simulink library "Steer_Rack_WheelByWire"  (R2025a)
settings: Solver=VariableStepAuto  StartTime=0.0  StopTime=10.0  RelTol=1e-3
undefined symbols (not defined in the file): Steer, Visual, X, Y, Z
libraries: fl_lib x15, sm_lib x11, nesl_utility x10, ee_lib x2, Driver_Systems x1, simulink_extras x1, sdl_lib x1, SteeringWheel x1, Vehicle_Inputs x1
Description:
  | Component of Simscape Vehicle Templates Library
  | 
  | Copyright 2018-2026 The MathWorks, Inc.
settings Model: Creator=smiller  LastModifiedBy=smiller
settings OptimizationCC: ReuseModelBlockBuffer=off
settings ModelReferenceCC: EnableRefExpFcnMdlSchedulingChecks=on
settings RTWCC: GPUComputeCapability=3.5

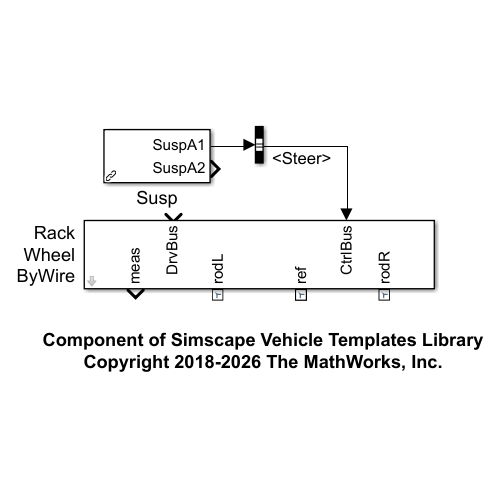
[thumbnail: Simulink's stored preview of the top-level diagram]
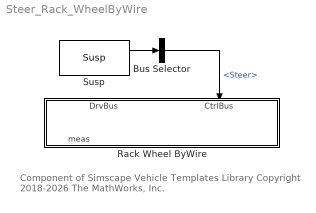
== system Steer_Rack_WheelByWire ==
  note: Component of Simscape Vehicle Templates Library
      | Copyright 2018-2026 The MathWorks, Inc.
  Bus Selector : BusSelector  OutputSignals=Steer
  Rack Wheel ByWire : Subsystem  Tag=PublishSubsystem  VariantControl=Rack  mask(Steer by Wire with Rack Actuation){hp_wheel=Steer.Wheel.sMount.Value, wheel_axis_incl=Steer.Wheel.aAxis.Value, hp_mt_rack=Steer.Rack.sMount.Value, hp_out_rack=Steer.Rack.sOutboard.Value, Wheel=Steer.Wheel, rack_mass=Steer.Rack.m.Value, whl2rack_filter=1/Steer.Rack.fActuatorCutoff.Value, clr_rack=Visual.SteeringRack.clr, opc_rack=Visual.part.opc, radius_rack=Visual.SteeringRack.rad, clr_connhp=Visual.hp.clr, opc_connhp=Visual.hp.opc, size_connhp=Visual.hp.rad, clr_wheel=Visual.SteeringWheel.clr, opc_wheel=Visual.part.opc, DriverHuman=Steer.DriverHuman, Kp_breakpoints=Steer.Control.KpTable.xRack.Value, Kp_values=Steer.Control.KpTable.Kp.Value, Ki=Steer.Control.Ki.Value, Kd=Steer.Control.Kd.Value, tFilt_xRack=1/Steer.Control.fRackxCutoff.Value, tFilt_deriv=1/Steer.Control.fErrDerCutoff.Value, nTrqSteer=Steer.Control.nSteerTrq.Value, vDC=Steer.vMotor.Value, mSteer_trq=Steer.MotorSteer.TorqueSpd.trq.Value, mSteer_spd=Steer.MotorSteer.TorqueSpd.w.Value, mSteer_tc=1/Steer.MotorSteer.fActuatorCutoff.Value, mSteer_J=Steer.MotorSteer.J.Value, mSteer_d=Steer.MotorSteer.D.Value, mRack_trq=Steer.MotorRack.TorqueSpd.trq.Value, mRack_spd=Steer.MotorRack.TorqueSpd.w.Value, mRack_tc=1/Steer.MotorRack.fActuatorCutoff.Value, mRack_J=Steer.MotorRack.J.Value, mRack_d=Steer.MotorRack.D.Value, kRackCompliance=Steer.Rack.kCompliance.Value, DRackCompliance=Steer.Rack.DCompliance.Value, rPinion=Steer.Rack.xPinionRadius.Value, DRack=Steer.Rack.DHousing.Value}
      mask prompts: hp_wheel "HP Wheel [xyz] (m)"; wheel_axis_incl "Wheel Axis Angle (rad)"; hp_mt_rack "HP Rack Mount [xyz] (m)"; hp_out_rack "HP Track Rod Inboard [xyz] (m)"; whl2rack_filter "Rack Motion Filter (sec)"; DriverHuman "Driver Human (structure)"; Kp_breakpoints "Kp Table, Rack position (m)"; Kp_values "Kp Table, Value"; Ki "Ki Controller Gain"; Kd "Kd Controller Gain"; tFilt_xRack "Rack Position Filter (sec)"; tFilt_deriv "Error Derivative Filter (sec)"; nTrqSteer "Gain, Steer Torque"; vDC "DC Voltage (V)"; mSteer_trq "Max Torque (N*m)"; mSteer_spd "Speeds (rpm)"; mSteer_tc "Torque Control Filter (sec)"; mSteer_J "Rotor Inertia (kg*m^2)"; mSteer_d "Rotor Damping (N*m/(m/s))"; mRack_trq "Max Torque (N*m)"; mRack_spd "Speeds (rpm)"; mRack_tc "Torque Control Filter (sec)"; mRack_J "Rotor Inertia (kg*m^2)"; mRack_d "Rotor Damping (N*m/(m/s))"; kRackCompliance "Rack Compliance Stiffness (N/m)"; DRackCompliance "Rack Compliance Damping (N/(m/s))"; rPinion "Pinion Radius (m)"; DRack "Rack Damping (N/(m/s))"
      mask help: Models steer by wire system. Steering wheel angle follows the target angle. Rack position is controlled by a motor The controller also commands a separate motor which applies torque to the steering wheel. This torque provides feedback to the driver concerning the force required to position the rack.
      mask TypeOptions hp_wheel:
      | Ref to Wheel/Transform
      | HP Wheel/TranslationCartesianOffset
      mask TypeOptions hp_mt_rack:
      | Ref to Rack/Transform
      | HP Rack/TranslationCartesianOffset
      mask TypeOptions hp_out_rack: Rack/hp_out
      mask TypeOptions rack_mass: Rack/rack_mass
      mask TypeOptions whl2rack_filter: Physical Signal/InputFilterTimeConstant
      mask TypeOptions clr_rack: Rack/clr_rack
      mask TypeOptions opc_rack: Rack/opc_rack
      mask TypeOptions radius_rack: Rack/radius_rack
      mask TypeOptions clr_connhp:
      | Ref to Rack/Vis
      | Rack
      | Housing/GraphicDiffuseColor
      mask TypeOptions opc_connhp:
      | Ref to Rack/Vis
      | Rack
      | Housing/GraphicOpacity
      mask TypeOptions size_connhp:
      | Ref to Rack/Vis
      | Rack
      | Housing/SphereRadius
      mask TypeOptions clr_wheel: Wheel/clr_wheel
      mask TypeOptions opc_wheel: Wheel/opc_wheel
      mask TypeOptions Kp_breakpoints: Motors/Kp_breakpoints
      mask TypeOptions Kp_values: Motors/Kp_values
      mask TypeOptions Ki: Motors/Ki
      mask TypeOptions Kd: Motors/Kd
      mask TypeOptions tFilt_xRack: Motors/tFilt_xRack
      mask TypeOptions tFilt_deriv: Motors/tFilt_deriv
      mask TypeOptions nTrqSteer: Motors/nTrqSteer
      mask TypeOptions vDC: Motors/vDC
      mask TypeOptions mSteer_trq: Motors/mSteer_trq
      mask TypeOptions mSteer_spd: Motors/mSteer_spd
      mask TypeOptions mSteer_tc: Motors/mSteer_tc
      mask TypeOptions mSteer_J: Motors/mSteer_J
      mask TypeOptions mSteer_d: Motors/mSteer_d
      mask TypeOptions mRack_trq: Motors/mRack_trq
      mask TypeOptions mRack_spd: Motors/mRack_spd
      mask TypeOptions mRack_tc: Motors/mRack_tc
      mask TypeOptions mRack_J: Motors/mRack_J
      mask TypeOptions mRack_d: Motors/mRack_d
      mask TypeOptions kRackCompliance: Motors/kRackCompliance
      mask TypeOptions DRackCompliance: Motors/DRackCompliance
      mask TypeOptions rPinion: Motors/rPinion
      mask TypeOptions DRack: Motors/DRack
      mask DialogControl cont_steer Prompt: Steer
      mask DialogControl grp_strparts Prompt: Parts
      mask DialogControl text_strparts_len Prompt: Length/Radius (m)
      mask DialogControl text_strparts_mass Prompt: Mass (kg)
      mask DialogControl text_strparts_wheel Prompt: Wheel
      mask DialogControl text_strparts_wheel_m Prompt: <CAD file>
      mask DialogControl text_strparts_rack Prompt: Rack
      mask DialogControl text_strparts_rack_len Prompt: <HP Rod Inboard>
      mask DialogControl grp_whl2rack Prompt: Wheel to Rack
      mask DialogControl cont_vis_steer Prompt: Visualization
      mask DialogControl text_steer_vis_clr Prompt: Color [RGB]
      mask DialogControl text_steer_vis_opc Prompt: Opac. (0-1)
      mask DialogControl text_steer_vis_size Prompt: Size (m)
      mask DialogControl text_steer_vis_rack Prompt: Rack
      mask DialogControl text_steer_vis_connhp Prompt: Connections, HP
      mask DialogControl text_steer_vis_wheel Prompt: Wheel
      mask DialogControl text_wheel_size Prompt: <CAD File>
      mask DialogControl cont_driver_human Prompt: Driver Human
      mask DialogControl cont_controller Prompt: Control
      mask DialogControl cont_motor Prompt: Motor
      mask DialogControl grp_steer Prompt: Steer
      mask DialogControl grp_rack Prompt: Rack
      mask DialogControl cont_rack Prompt: Rack
  Susp : Vehicle_Inputs/Control Bus/Susp  SystemSampleTime=-1  VariantActivationTime=update diagram  EmptyChoice=off  PassThrough=off  PassThroughVariantControl=(default)  EmptyChoiceVariantControl=(default)  AllowFlexibleInterface=on  Latency=0  AutoFrameSizeCalculation=off
  wires:
  Bus Selector/1 -> Rack Wheel ByWire/2(CtrlBus)  "<Steer>"
  Susp/1 -> Bus Selector/1

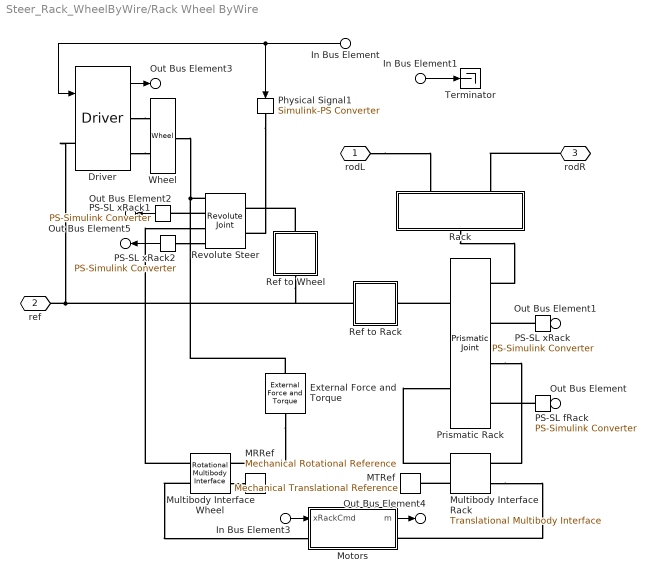
== system Steer_Rack_WheelByWire/Rack Wheel ByWire ==
  In Bus Element1 : Inport  PortName=DrvBus  Element=aSteerWheel
  In Bus Element : Inport  Port=2  PortName=CtrlBus  Element=aSteerWheel
  In Bus Element3 : Inport  Port=2  PortName=CtrlBus  Element=xRack
  Driver : Driver_Systems/Driver  LabelModeActiveChoice=Human  DriverHuman=DriverHuman  VariantLabel=DriverHuman.class.Value
      settings: AttributesFormatString=%<LabelModeActiveChoice>
  External Force and Torque : sm_lib/Forces and Torques/External Force and Torque  EnableForceX=off  EnableForceY=off  EnableForceZ=off  EnableForce=off  ForceResolutionFrame=AttachedFrame  EnableTorqueX=off  EnableTorqueY=off  EnableTorqueZ=on  EnableTorque=off  TorqueResolutionFrame=AttachedFrame
  MRRef : fl_lib/Mechanical/Rotational Elements/Mechanical Rotational Reference
  MTRef : fl_lib/Mechanical/Translational Elements/Mechanical Translational Reference
  Motors : Subsystem  mask{Kp_breakpoints=Kp_breakpoints, Kp_values=Kp_values, Ki=Ki, Kd=Kd, tFilt_deriv=tFilt_deriv, tFilt_xRack=tFilt_xRack, nTrqSteer=nTrqSteer, vDC=vDC, mSteer_trq=mSteer_trq, mSteer_spd=mSteer_spd, mSteer_tc=mSteer_tc, mSteer_J=mSteer_J, mSteer_d=mSteer_d, mRack_trq=mRack_trq, mRack_spd=mRack_spd, mRack_tc=mRack_tc, mRack_J=mRack_J, mRack_d=mRack_d, rPinion=rPinion, kRackCompliance=kRackCompliance, DRackCompliance=DRackCompliance, DRack=DRack}
      mask prompts: Kp_breakpoints "Kp Table, Rack position (m)"; Kp_values "Kp Table, Value"; Ki "Ki Controller Gain"; Kd "Kd Controller Gain"; tFilt_deriv "Filter Constant, Error Derivative"; tFilt_xRack "Filter Constant Rack Position"; nTrqSteer "Gain, Steer Torque"; vDC "DC Voltage (V)"; mSteer_trq "Max Torque (N*m)"; mSteer_spd "Speeds (rpm)"; mSteer_tc "Torque control time constant (sec)"; mSteer_J "Rotor Inertia (kg*m^2)"; mSteer_d "Rotor damping"; mRack_trq "Max Torque (N*m)"; mRack_spd "Speeds (rpm)"; mRack_tc "Torque control time constant (sec)"; mRack_J "Rotor Inertia (kg*m^2)"; mRack_d "Rotor damping"; rPinion "Pinion Radius (m)"; kRackCompliance "Rack Compliance Stiffness (N/m)"; DRackCompliance "Rack Compliance Damping (N/(m/s))"; DRack "Rack Damping (N/(m/s))"
      mask TypeOptions Kp_breakpoints: Control/Kp_breakpoints
      mask TypeOptions Kp_values: Control/Kp_values
      mask TypeOptions Ki: Control/Ki
      mask TypeOptions Kd: Control/Kd
      mask TypeOptions tFilt_deriv: Control/tFilt_deriv
      mask TypeOptions tFilt_xRack: Control/tFilt_xRack
      mask TypeOptions nTrqSteer: Control/nTrqSteer
      mask TypeOptions vDC:
      | DC
      | Voltage
      | Source/v0
      mask TypeOptions mSteer_trq:
      | Motor
      | Steer/T_t
      mask TypeOptions mSteer_spd:
      | Motor
      | Steer/w_t
      mask TypeOptions mSteer_tc:
      | Motor
      | Steer/Tc
      mask TypeOptions mSteer_J:
      | Motor
      | Steer/J
      mask TypeOptions mSteer_d:
      | Motor
      | Steer/lam
      mask TypeOptions mRack_trq:
      | Motor
      | Rack/T_t
      mask TypeOptions mRack_spd:
      | Motor
      | Rack/w_t
      mask TypeOptions mRack_tc:
      | Motor
      | Rack/Tc
      mask TypeOptions mRack_J:
      | Motor
      | Rack/J
      mask TypeOptions mRack_d:
      | Motor
      | Rack/lam
      mask TypeOptions rPinion: Wheel and Axle/R
      mask TypeOptions kRackCompliance:
      | Compliance
      | Spring/spr_rate
      mask TypeOptions DRackCompliance:
      | Compliance
      | Damper/D
      mask TypeOptions DRack: Rack Damper/D
      mask DialogControl tab_control Prompt: Control
      mask DialogControl tab_motor Prompt: Motor
      mask DialogControl grp_steer Prompt: Steer
      mask DialogControl grp_rack Prompt: Rack
      mask DialogControl cont_rack Prompt: Rack
  Multibody Interface Rack : fl_lib/Mechanical/Multibody Interfaces/Translational Multibody Interface
  Multibody Interface Wheel : fl_lib/Mechanical/Multibody Interfaces/Rotational Multibody Interface
  PS-SL fRack : nesl_utility/PS-Simulink Converter  PhysicalDomain=network_engine_domain  SubClassName=ps_output  LeftPortType=input  RightPortType=output  PseudoPeriodic=off  Frequencies=[]  VectorFormat=1-D array  Unit=1  AffineConversion=off
  PS-SL xRack : nesl_utility/PS-Simulink Converter  PhysicalDomain=network_engine_domain  SubClassName=ps_output  LeftPortType=input  RightPortType=output  PseudoPeriodic=off  Frequencies=[]  VectorFormat=1-D array  Unit=1  AffineConversion=off
  PS-SL xRack1 : nesl_utility/PS-Simulink Converter  PhysicalDomain=network_engine_domain  SubClassName=ps_output  LeftPortType=input  RightPortType=output  PseudoPeriodic=off  Frequencies=[]  VectorFormat=1-D array  Unit=rad  AffineConversion=off
  PS-SL xRack2 : nesl_utility/PS-Simulink Converter  PhysicalDomain=network_engine_domain  SubClassName=ps_output  LeftPortType=input  RightPortType=output  PseudoPeriodic=off  Frequencies=[]  VectorFormat=1-D array  Unit=N*m  AffineConversion=off
  Physical Signal1 : nesl_utility/Simulink-PS Converter  PhysicalDomain=network_engine_domain  SubClassName=ps_input  LeftPortType=input  RightPortType=output  PseudoPeriodic=off  Frequencies=[]  NoiseDistribution=none  NoiseParameters=[]  Unit=rad  AffineConversion=off  FilteringAndDerivatives=filter  SimscapeFilterOrder=2  InputFilterTimeConstant=whl2rack_filter  UdotUserProvided=0
      settings: AttributesFormatString=|
      | Filter Time Constant
      | %<InputFilterTimeConstant> sec
  Prismatic Rack : sm_lib/Joints/Prismatic Joint  JointMode=Normal  CompositeWrenchDir=FollowerOnBase  CompositeWrenchFrame=BaseFrame  SenseConstraintForce=off  SenseConstraintTorque=off  SenseTotalForce=off  SenseTotalTorque=off  PositionTargetSpecify=on  PositionTargetPriority=Low  PositionTargetValue=0  PositionTargetValueUnits=m  VelocityTargetSpecify=off  VelocityTargetPriority=High  VelocityTargetValue=0  VelocityTargetValueUnits=m/s  EquilibriumPosition=0  EquilibriumPositionUnits=m  SpringStiffness=0  SpringStiffnessUnits=N/m  DampingCoefficient=1e2*0  DampingCoefficientUnits=N/(m/s)  LowerLimitSpecify=off  LowerLimitBound=-1  LowerLimitBoundUnits=m  LowerLimitStiffness=1e6  LowerLimitStiffnessUnits=N/m  LowerLimitDamping=1e3  LowerLimitDampingUnits=N/(m/s)  LowerLimitTransitionRegionWidth=1e-4  LowerLimitTransitionRegionWidthUnits=m  UpperLimitSpecify=off  UpperLimitBound=1  UpperLimitBoundUnits=m  UpperLimitStiffness=1e6  UpperLimitStiffnessUnits=N/m  UpperLimitDamping=1e3  UpperLimitDampingUnits=N/(m/s)  UpperLimitTransitionRegionWidth=1e-4  UpperLimitTransitionRegionWidthUnits=m  TorqueActuationMode=InputTorque  MotionActuationMode=ComputedMotion  SensePosition=on  SenseVelocity=on  SenseAcceleration=off  SenseTorqueForce=on  SenseLowerLimitTorqueForce=off  SenseUpperLimitTorqueForce=off
  Rack : Subsystem  mask{hp_out=hp_out_rack, rack_mass=rack_mass, clr_rack=clr_rack, opc_rack=opc_rack, radius_rack=radius_rack}
      mask prompts: hp_out "HP Track Rod Inboard [xyz] (m)"; rack_mass "Mass (kg)"
      mask init:
      | rack_length = norm(hp_out-hp_out.*[1 -1 1]);
      mask TypeOptions rack_mass: Rack/Mass
      mask TypeOptions clr_rack: Rack/GraphicDiffuseColor
      mask TypeOptions opc_rack: Rack/GraphicOpacity
      mask TypeOptions radius_rack: Rack/CylinderRadius
      mask DialogControl cont_rack Prompt: Rack
      mask DialogControl text_rack_clr Prompt: Color [RGB]
      mask DialogControl text_rack_opc Prompt: Opac. (0-1)
      mask DialogControl text_rack_size Prompt: Size (m)
      mask DialogControl text_rack_rack Prompt: Rack
  Ref to Rack : Subsystem
  Ref to Wheel : Subsystem
  Revolute Steer : sm_lib/Joints/Revolute Joint  JointMode=Normal  CompositeWrenchDir=FollowerOnBase  CompositeWrenchFrame=BaseFrame  SenseConstraintForce=off  SenseConstraintTorque=off  SenseTotalForce=off  SenseTotalTorque=off  PositionTargetSpecify=on  PositionTargetPriority=High  PositionTargetValue=0  PositionTargetValueUnits=deg  VelocityTargetSpecify=off  VelocityTargetPriority=High  VelocityTargetValue=0  VelocityTargetValueUnits=deg/s  EquilibriumPosition=0  EquilibriumPositionUnits=deg  SpringStiffness=0  SpringStiffnessUnits=N*m/deg  DampingCoefficient=0  DampingCoefficientUnits=N*m/(deg/s)  LowerLimitSpecify=off  LowerLimitBound=-90  LowerLimitBoundUnits=deg  LowerLimitStiffness=1e4  LowerLimitStiffnessUnits=N*m/deg  LowerLimitDamping=10  LowerLimitDampingUnits=N*m/(deg/s)  LowerLimitTransitionRegionWidth=0.1  LowerLimitTransitionRegionWidthUnits=deg  UpperLimitSpecify=off  UpperLimitBound=90  UpperLimitBoundUnits=deg  UpperLimitStiffness=1e4  UpperLimitStiffnessUnits=N*m/deg  UpperLimitDamping=10  UpperLimitDampingUnits=N*m/(deg/s)  UpperLimitTransitionRegionWidth=0.1  UpperLimitTransitionRegionWidthUnits=deg  TorqueActuationMode=ComputedTorque  MotionActuationMode=InputMotion  SensePosition=on  SenseVelocity=on  SenseAcceleration=off  SenseTorqueForce=on  SenseLowerLimitTorqueForce=off  SenseUpperLimitTorqueForce=off
  Terminator : Terminator
  Wheel : SteeringWheel/Wheel  LabelModeActiveChoice=Sedan  VariantLabel=Wheel.class.Value
  rodL : PMIOPort  Side=Right
  ref : PMIOPort  Port=2  Side=Right
  rodR : PMIOPort  Port=3  Side=Right
  Out Bus Element : Outport  VectorParamsAs1DForOutWhenUnconnected=off  PortName=meas  Element=FRack
  Out Bus Element1 : Outport  VectorParamsAs1DForOutWhenUnconnected=off  PortName=meas  Element=xRack
  Out Bus Element2 : Outport  VectorParamsAs1DForOutWhenUnconnected=off  PortName=meas  Element=aWheel
  Out Bus Element3 : Outport  VectorParamsAs1DForOutWhenUnconnected=off  PortName=meas  Element=Driver
  Out Bus Element4 : Outport  VectorParamsAs1DForOutWhenUnconnected=off  PortName=meas  Element=Motor
  Out Bus Element5 : Outport  VectorParamsAs1DForOutWhenUnconnected=off  PortName=meas  Element=trqWheel
  wires:
  In Bus Element1/1 -> Terminator/1
  Driver/1 -> Out Bus Element3/1
  PS-SL xRack1/1 -> Out Bus Element2/1
  In Bus Element/1 -> Driver/1, Physical Signal1/1
  PS-SL fRack/1 -> Out Bus Element/1
  PS-SL xRack/1 -> Out Bus Element1/1
  In Bus Element3/1 -> Motors/1(xRackCmd)
  Motors/1(m) -> Out Bus Element4/1
  PS-SL xRack2/1 -> Out Bus Element5/1
  connections:
  Driver/RConn2 -- Wheel/RConn2
  Driver/RConn1 -- Wheel/RConn1
  Multibody Interface Wheel/RConn1 -- Revolute Steer/RConn3
  rodR/RConn1 -- Rack/LConn2
  rodL/RConn1 -- Rack/LConn1
  Prismatic Rack/LConn1 -- Ref to Rack/RConn1
  Ref to Wheel/RConn1 -- Revolute Steer/LConn1
  Wheel/LConn1 -- Revolute Steer/RConn1 -- External Force and Torque/RConn1
  PS-SL xRack/LConn1 -- Prismatic Rack/RConn2
  Rack/RConn1 -- Prismatic Rack/RConn1
  Driver/LConn1 -- ref/RConn1 -- Ref to Rack/LConn1 -- Ref to Wheel/LConn1
  PS-SL fRack/LConn1 -- Prismatic Rack/RConn4
  Multibody Interface Wheel/RConn2 -- Motors/LConn1
  External Force and Torque/LConn1 -- Multibody Interface Wheel/LConn1
  Multibody Interface Wheel/LConn2 -- MRRef/LConn1
  Multibody Interface Rack/RConn2 -- Motors/RConn1
  Prismatic Rack/RConn3 -- Multibody Interface Rack/RConn1
  Multibody Interface Rack/LConn1 -- Prismatic Rack/LConn2
  Multibody Interface Rack/LConn2 -- MTRef/LConn1
  Physical Signal1/RConn1 -- Revolute Steer/LConn2
  Revolute Steer/RConn2 -- PS-SL xRack1/LConn1
  PS-SL xRack2/LConn1 -- Revolute Steer/RConn4

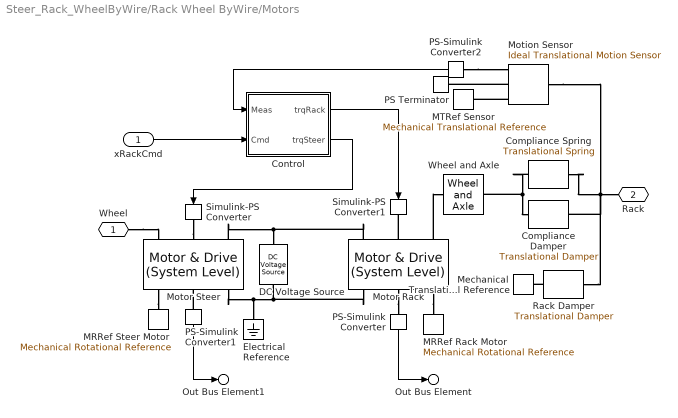
== system Steer_Rack_WheelByWire/Rack Wheel ByWire/Motors ==
  xRackCmd : Inport
  Compliance Damper : fl_lib/Mechanical/Translational Elements/Translational Damper  D=DRackCompliance N*s/m  v_specify=off  v_priority=None  v=0 m/s  v_nominal_specify=off  v_nominal_value=1  v_nominal_unit=m/s  f_specify=off  f_priority=None  f=0 N  f_nominal_specify=off  f_nominal_value=1  f_nominal_unit=N
  Compliance Spring : fl_lib/Mechanical/Translational Elements/Translational Spring  spr_rate=kRackCompliance N/m  v_specify=off  v_priority=None  v=0 m/s  v_nominal_specify=off  v_nominal_value=1  v_nominal_unit=m/s  f_specify=off  f_priority=None  f=0 N  f_nominal_specify=off  f_nominal_value=1  f_nominal_unit=N  x_specify=off  x_priority=High  x=0 m  x_nominal_specify=off  x_nominal_value=1  x_nominal_unit=m
  Control : Subsystem  mask{Kp_breakpoints=Kp_breakpoints, Kp_values=Kp_values, Ki=Ki, Kd=Kd, tFilt_xRack=tFilt_xRack, tFilt_deriv=tFilt_deriv, nTrqSteer=nTrqSteer}
      mask prompts: Kp_breakpoints "Kp Table, Rack position (m)"; Kp_values "Kp Table, Value"; Ki "Ki Controller Gain"; Kd "Kd Controller Gain"; tFilt_xRack "Filter Constant Rack Position"; tFilt_deriv "Filter Constant, Error Derivative"; nTrqSteer "Gain, Steer Torque"
      mask TypeOptions Kp_breakpoints: Kp/BreakpointsForDimension1
      mask TypeOptions Kp_values: Kp/Table
      mask TypeOptions Ki: Ki/Gain
      mask TypeOptions Kd: Kd/Gain
      mask TypeOptions nTrqSteer: Steer Torque Factor/Value
  DC Voltage Source : fl_lib/Electrical/Electrical Sources/DC Voltage Source  v0=vDC V
  Electrical Reference : fl_lib/Electrical/Electrical Elements/Electrical Reference
  MRRef Rack Motor : fl_lib/Mechanical/Rotational Elements/Mechanical Rotational Reference
  MRRef Steer Motor : fl_lib/Mechanical/Rotational Elements/Mechanical Rotational Reference
  MTRef Sensor : fl_lib/Mechanical/Translational Elements/Mechanical Translational Reference
  Mechanical Translational Reference : fl_lib/Mechanical/Translational Elements/Mechanical Translational Reference
  Motion Sensor : fl_lib/Mechanical/Mechanical Sensors/Ideal Translational Motion Sensor  reference=foundation.enum.MeasurementReference.difference  acceleration_port=false  velocity_port=true  position_port=true  offset=0 m
  Motor Rack : ee_lib/Electromechanical/Motor & Drive (System Level)  torque_speed_param=ee.enum.electromech.envelope.tabulated  overtorque_param=ee.enum.electromech.overtorque.no  T_t=mRack_trq N*m  T_t_intermittent=[.36, .32, .28, 0] N*m  T_t_2D=[.09, .09, .09; .08, .08, .08; .07, .07, .07; 0, 0, 0] N*m  T_t_intermittent_2D=[.36, .36, .36; .32, .32, .32; .28, .28, .28; 0, 0, 0] N*m  w_t=mRack_spd rpm  vdc_t=[6, 12, 24] V  torque_max=0.1 N*m  power_max=30 W  torque_max_intermittent=0.4 N*m  power_max_intermittent=120 W  time_overtorque=30 s  time_recover=60 s  Tc=mRack_tc s  EnableSwitch=simscape.enum.onoff.off  losses_param=1  eff=100  w_eff=1800 rpm  T_eff=180 N*m  Piron=0 W  Pbase=0 W  w_eff_vec=[-8000, -4000, 0, 4000, 8000] rpm  T_eff_vec=[0, .03, .06, .09] N*m  v_eff_vec=[100, 250, 400] V  losses_mat=[1.49, 1.67, 2.21, 3.1; .42, .69, 1.14, 2.03; .06, .24, .78, 1.68; .42, .69, 1.14, 2.03; 1.49, 1.67, 2.21, 3.1] W  efficiency_mat=[95, 95, 95, 95; 95, 95, 95, 95; 95, 95, 95, 95; 95, 95, 95, 95; 95, 95, 95, 95]  losses_mat_3D=ones(5, 4, 3) W  efficiency_mat_3D=95 * ones(5, 4, 3)  Res=0 Ohm  J=mRack_J kg*m^2  lam=mRack_d N*m*s/rad  speed0=0 rpm  faulted_specify=off  faulted_priority=None  faulted=0  faulted_nominal_specify=off  faulted_nominal_value=1  faulted_nominal_unit=1  isSwitchedOff_specify=off  isSwitchedOff_priority=None  isSwitchedOff=0  isSwitchedOff_nominal_specify=off  isSwitchedOff_nominal_value=1  isSwitchedOff_nominal_unit=1  torqueLimitContinuous_specify=off  torqueLimitContinuous_priority=None  torqueLimitContinuous=0 N*m  torqueLimitContinuous_nominal_specify=off  torqueLimitContinuous_nominal_value=1  torqueLimitContinuous_nominal_unit=N*m  alpha=3.93e-3 1/K  Tmeas=25 degC  Tmeas2=125 degC  losses_mat_T2=[1.49, 1.74, 2.49, 3.74; .42, .67, 1.42, 2.67; .06, .31, 1.06, 2.31; .42, .67, 1.42, 2.67; 1.49, 1.74, 2.49, 3.74] W  efficiency_mat_T2=[95, 95, 95, 95; 95, 95, 95, 95; 95, 95, 95, 95; 95, 95, 95, 95; 95, 95, 95, 95]  losses_mat_3D_T2=ones(5, 4, 3) W  efficiency_mat_3D_T2=95 * ones(5, 4, 3)  thermal_mass=100 J/K  initial_temperature=25 degC
  Motor Steer : ee_lib/Electromechanical/Motor & Drive (System Level)  torque_speed_param=ee.enum.electromech.envelope.tabulated  overtorque_param=ee.enum.electromech.overtorque.no  T_t=mSteer_trq N*m  T_t_intermittent=[.36, .32, .28, 0] N*m  T_t_2D=[.09, .09, .09; .08, .08, .08; .07, .07, .07; 0, 0, 0] N*m  T_t_intermittent_2D=[.36, .36, .36; .32, .32, .32; .28, .28, .28; 0, 0, 0] N*m  w_t=mSteer_spd rpm  vdc_t=[6, 12, 24] V  torque_max=0.1 N*m  power_max=30 W  torque_max_intermittent=0.4 N*m  power_max_intermittent=120 W  time_overtorque=30 s  time_recover=60 s  Tc=mSteer_tc s  EnableSwitch=simscape.enum.onoff.off  losses_param=1  eff=100  w_eff=3750 rpm  T_eff=180 N*m  Piron=0 W  Pbase=0 W  w_eff_vec=[-8000, -4000, 0, 4000, 8000] rpm  T_eff_vec=[0, .03, .06, .09] N*m  v_eff_vec=[100, 250, 400] V  losses_mat=[1.49, 1.67, 2.21, 3.1; .42, .69, 1.14, 2.03; .06, .24, .78, 1.68; .42, .69, 1.14, 2.03; 1.49, 1.67, 2.21, 3.1] W  efficiency_mat=[95, 95, 95, 95; 95, 95, 95, 95; 95, 95, 95, 95; 95, 95, 95, 95; 95, 95, 95, 95]  losses_mat_3D=ones(5, 4, 3) W  efficiency_mat_3D=95 * ones(5, 4, 3)  Res=0 Ohm  J=mSteer_J kg*m^2  lam=mSteer_d N*m*s/rad  speed0=0 rpm  faulted_specify=off  faulted_priority=None  faulted=0  faulted_nominal_specify=off  faulted_nominal_value=1  faulted_nominal_unit=1  isSwitchedOff_specify=off  isSwitchedOff_priority=None  isSwitchedOff=0  isSwitchedOff_nominal_specify=off  isSwitchedOff_nominal_value=1  isSwitchedOff_nominal_unit=1  torqueLimitContinuous_specify=off  torqueLimitContinuous_priority=None  torqueLimitContinuous=0 N*m  torqueLimitContinuous_nominal_specify=off  torqueLimitContinuous_nominal_value=1  torqueLimitContinuous_nominal_unit=N*m  alpha=3.93e-3 1/K  Tmeas=25 degC  Tmeas2=125 degC  losses_mat_T2=[1.49, 1.74, 2.49, 3.74; .42, .67, 1.42, 2.67; .06, .31, 1.06, 2.31; .42, .67, 1.42, 2.67; 1.49, 1.74, 2.49, 3.74] W  efficiency_mat_T2=[95, 95, 95, 95; 95, 95, 95, 95; 95, 95, 95, 95; 95, 95, 95, 95; 95, 95, 95, 95]  losses_mat_3D_T2=ones(5, 4, 3) W  efficiency_mat_3D_T2=95 * ones(5, 4, 3)  thermal_mass=100 J/K  initial_temperature=25 degC
  PS Terminator : fl_lib/Physical Signals/Sinks/PS Terminator
  PS-Simulink Converter : nesl_utility/PS-Simulink Converter  PhysicalDomain=network_engine_domain  SubClassName=ps_output  LeftPortType=input  RightPortType=output  PseudoPeriodic=off  Frequencies=[]  VectorFormat=inherit  Unit=inherit  AffineConversion=off
  PS-Simulink Converter1 : nesl_utility/PS-Simulink Converter  PhysicalDomain=network_engine_domain  SubClassName=ps_output  LeftPortType=input  RightPortType=output  PseudoPeriodic=off  Frequencies=[]  VectorFormat=inherit  Unit=inherit  AffineConversion=off
  PS-Simulink Converter2 : nesl_utility/PS-Simulink Converter  PhysicalDomain=network_engine_domain  SubClassName=ps_output  LeftPortType=input  RightPortType=output  PseudoPeriodic=off  Frequencies=[]  VectorFormat=inherit  Unit=inherit  AffineConversion=off
  Rack Damper : sdl_lib/Couplings & Drives/Springs & Dampers/Translational Damper  D=DRack N*s/m  thermal_port=simscape.enum.thermaleffects.omit  thermal_mass=50 kJ/K  temperature_specify=off  temperature_priority=High  temperature=300 K  temperature_nominal_specify=off  temperature_nominal_value=1  temperature_nominal_unit=K
  Simulink-PS Converter : nesl_utility/Simulink-PS Converter  PhysicalDomain=network_engine_domain  SubClassName=ps_input  LeftPortType=input  RightPortType=output  PseudoPeriodic=off  Frequencies=[]  NoiseDistribution=none  NoiseParameters=[]  Unit=1  AffineConversion=off  FilteringAndDerivatives=provide  SimscapeFilterOrder=1  InputFilterTimeConstant=0.001  UdotUserProvided=0
  Simulink-PS Converter1 : nesl_utility/Simulink-PS Converter  PhysicalDomain=network_engine_domain  SubClassName=ps_input  LeftPortType=input  RightPortType=output  PseudoPeriodic=off  Frequencies=[]  NoiseDistribution=none  NoiseParameters=[]  Unit=1  AffineConversion=off  FilteringAndDerivatives=provide  SimscapeFilterOrder=1  InputFilterTimeConstant=0.001  UdotUserProvided=0
  Wheel and Axle : fl_lib/Mechanical/Mechanisms/Wheel and Axle  R=rPinion m  or=1  t_specify=off  t_priority=None  t=0 N*m  t_nominal_specify=off  t_nominal_value=1  t_nominal_unit=N*m  f_specify=off  f_priority=None  f=0 N  f_nominal_specify=off  f_nominal_value=1  f_nominal_unit=N
  Wheel : PMIOPort  Side=Left
  Rack : PMIOPort  Port=2  Side=Right
  Out Bus Element : Outport  PortName=m  Element=Rack.w
  Out Bus Element1 : Outport  PortName=m  Element=Steer.w
  wires:
  Control/2(trqSteer) -> Simulink-PS Converter/1
  Control/1(trqRack) -> Simulink-PS Converter1/1
  PS-Simulink Converter/1 -> Out Bus Element/1
  PS-Simulink Converter1/1 -> Out Bus Element1/1
  xRackCmd/1 -> Control/2(Cmd)
  PS-Simulink Converter2/1 -> Control/1(Meas)
  connections:
  Motor Steer/LConn1 -- Motor Rack/LConn1 -- DC Voltage Source/LConn1
  Motor Rack/LConn3 -- Wheel and Axle/LConn1
  Motor Rack/RConn3 -- MRRef Rack Motor/LConn1
  Simulink-PS Converter/RConn1 -- Motor Steer/LConn2
  Motor Steer/RConn1 -- Motor Rack/RConn1 -- DC Voltage Source/RConn1 -- Electrical Reference/LConn1
  Compliance Spring/RConn1 -- Compliance Damper/RConn1 -- Wheel and Axle/RConn1
  Motor Rack/LConn2 -- Simulink-PS Converter1/RConn1
  PS-Simulink Converter1/LConn1 -- Motor Steer/RConn2
  Motor Steer/RConn3 -- MRRef Steer Motor/LConn1
  Motor Rack/RConn2 -- PS-Simulink Converter/LConn1
  Wheel/RConn1 -- Motor Steer/LConn3
  Motion Sensor/RConn1 -- MTRef Sensor/LConn1
  PS-Simulink Converter2/LConn1 -- Motion Sensor/RConn3
  Motion Sensor/RConn2 -- PS Terminator/LConn1
  Motion Sensor/LConn1 -- Compliance Spring/LConn1 -- Compliance Damper/LConn1 -- Rack Damper/LConn1 -- Rack/RConn1
  Rack Damper/RConn1 -- Mechanical Translational Reference/LConn1

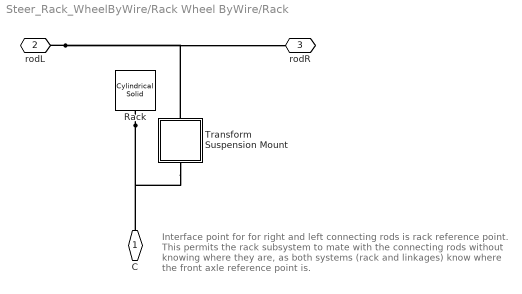
== system Steer_Rack_WheelByWire/Rack Wheel ByWire/Rack ==
  note: Interface point for for right and left connecting rods is rack reference point. This permits the rack subsystem to mate with the connecting rods without knowing where they are, as both systems (rack and linkages) know where the front axle reference point is.
  Rack : sm_lib/Body Elements/Cylindrical Solid  CylinderRadius=radius_rack  CylinderRadiusUnits=m  CylinderLength=rack_length  CylinderLengthUnits=m  ExportEntireGeometry=off  InertiaType=CalculateFromGeometry  BasedOnType=Mass  Density=7000  DensityUnits=kg/m^3  Mass=rack_mass  MassUnits=kg  CenterOfMass=[0 0 0]  CenterOfMassUnits=m  MomentsOfInertia=[1 1 1]  MomentsOfInertiaUnits=kg*m^2  ProductsOfInertia=[0 0 0]  ProductsOfInertiaUnits=kg*m^2  GraphicType=FromGeometry  MarkerShape=Sphere  MarkerSize=10  GraphicVisPropType=SimpleVisualProperties  GraphicDiffuseColor=clr_rack  GraphicOpacity=opc_rack  GraphicSpecularColor=[0.5 0.5 0.5 1.0]  GraphicAmbientColor=[0.15 0.15 0.15 1.0]  GraphicEmissiveColor=[0.0 0.0 0.0 1.0]  GraphicShininess=75  DoExposeReferenceFrame=on  SerializedFrames=<Frames/>
  Transform Suspension Mount : Subsystem
  C : PMIOPort  Side=Right
  rodL : PMIOPort  Port=2  Side=Left
  rodR : PMIOPort  Port=3  Side=Left
  connections:
  rodL/RConn1 -- rodR/RConn1 -- Transform Suspension Mount/LConn1
  Rack/RConn1 -- Transform Suspension Mount/RConn1 -- C/RConn1

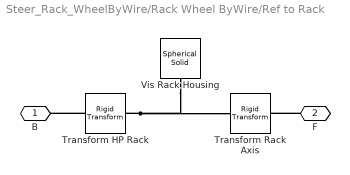
== system Steer_Rack_WheelByWire/Rack Wheel ByWire/Ref to Rack ==
  Transform HP Rack : sm_lib/Frames and Transforms/Rigid Transform  RotationMethod=None  FollAlignAxisA=+X  BaseAlignAxisA=+Y  FollAlignAxisB=+Y  BaseAlignAxisB=+Z  RotationStandardAxis=+Z  RotationAngle=0.0  RotationAngleUnits=deg  RotationArbitraryAxis=[0 0 1]  RotationSequenceAxes=FollowerAxes  RotationSequence=XYX  RotationSequenceAngles=[0 0 0]  RotationSequenceAnglesUnits=deg  RotationMatrix=[1 0 0; 0 1 0; 0 0 1]  Quaternion=[1 0 0 0]  TranslationMethod=Cartesian  TranslationCartesianOffset=hp_mt_rack  TranslationCartesianOffsetUnits=m  TranslationStandardAxis=+Z  TranslationStandardOffset=0  TranslationStandardOffsetUnits=m  TranslationROffset=0  TranslationROffsetUnits=m  TranslationThetaOffset=0  TranslationThetaOffsetUnits=deg  TranslationZOffset=0  TranslationZOffsetUnits=m
  Transform Rack Axis : sm_lib/Frames and Transforms/Rigid Transform  RotationMethod=AlignedAxes  FollAlignAxisA=+Y  BaseAlignAxisA=-Z  FollAlignAxisB=+X  BaseAlignAxisB=+X  RotationStandardAxis=+Z  RotationAngle=0  RotationAngleUnits=deg  RotationArbitraryAxis=[0 0 1]  RotationSequenceAxes=FollowerAxes  RotationSequence=XYX  RotationSequenceAngles=[0 0 0]  RotationSequenceAnglesUnits=deg  RotationMatrix=[0 0 -1;0 1 0;1 0 0]  Quaternion=[1 0 0 0]  TranslationMethod=None  TranslationCartesianOffset=[0 0 0]  TranslationCartesianOffsetUnits=m  TranslationStandardAxis=+Z  TranslationStandardOffset=0  TranslationStandardOffsetUnits=m  TranslationROffset=0  TranslationROffsetUnits=m  TranslationThetaOffset=0  TranslationThetaOffsetUnits=deg  TranslationZOffset=0  TranslationZOffsetUnits=m
  Vis Rack Housing : sm_lib/Body Elements/Spherical Solid  SphereRadius=size_connhp  SphereRadiusUnits=m  ExportEntireGeometry=off  InertiaType=CalculateFromGeometry  BasedOnType=Density  Density=1000  DensityUnits=kg/m^3  Mass=1  MassUnits=kg  CenterOfMass=[0 0 0]  CenterOfMassUnits=m  MomentsOfInertia=[1 1 1]  MomentsOfInertiaUnits=kg*m^2  ProductsOfInertia=[0 0 0]  ProductsOfInertiaUnits=kg*m^2  GraphicType=FromGeometry  MarkerShape=Sphere  MarkerSize=10  GraphicVisPropType=SimpleVisualProperties  GraphicDiffuseColor=clr_connhp  GraphicOpacity=opc_connhp  GraphicSpecularColor=[0.5 0.5 0.5 1.0]  GraphicAmbientColor=[0.15 0.15 0.15 1.0]  GraphicEmissiveColor=[0.0 0.0 0.0 1.0]  GraphicShininess=75  DoExposeReferenceFrame=on  SerializedFrames=<Frames/>
  B : PMIOPort  Side=Left
  F : PMIOPort  Port=2  Side=Right
  connections:
  F/RConn1 -- Transform Rack Axis/RConn1
  Transform HP Rack/LConn1 -- B/RConn1
  Transform HP Rack/RConn1 -- Transform Rack Axis/LConn1 -- Vis Rack Housing/RConn1

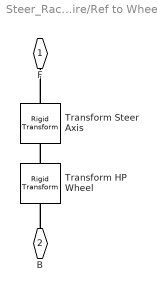
== system Steer_Rack_WheelByWire/Rack Wheel ByWire/Ref to Wheel ==
  Transform HP Wheel : sm_lib/Frames and Transforms/Rigid Transform  RotationMethod=None  FollAlignAxisA=+X  BaseAlignAxisA=+Y  FollAlignAxisB=+Y  BaseAlignAxisB=+Z  RotationStandardAxis=+Z  RotationAngle=0.0  RotationAngleUnits=deg  RotationArbitraryAxis=[0 0 1]  RotationSequenceAxes=FollowerAxes  RotationSequence=XYX  RotationSequenceAngles=[0 0 0]  RotationSequenceAnglesUnits=deg  RotationMatrix=[1 0 0; 0 1 0; 0 0 1]  Quaternion=[1 0 0 0]  TranslationMethod=Cartesian  TranslationCartesianOffset=hp_wheel  TranslationCartesianOffsetUnits=m  TranslationStandardAxis=+Z  TranslationStandardOffset=0  TranslationStandardOffsetUnits=m  TranslationROffset=0  TranslationROffsetUnits=m  TranslationThetaOffset=0  TranslationThetaOffsetUnits=deg  TranslationZOffset=0  TranslationZOffsetUnits=m
  Transform Steer Axis : sm_lib/Frames and Transforms/Rigid Transform  RotationMethod=StandardAxis  FollAlignAxisA=+X  BaseAlignAxisA=+Y  FollAlignAxisB=+Y  BaseAlignAxisB=+Z  RotationStandardAxis=+Y  RotationAngle=-pi/2+wheel_axis_incl  RotationAngleUnits=rad  RotationArbitraryAxis=[0 0 1]  RotationSequenceAxes=FollowerAxes  RotationSequence=XYX  RotationSequenceAngles=[0 0 0]  RotationSequenceAnglesUnits=deg  RotationMatrix=[1 0 0; 0 1 0; 0 0 1]  Quaternion=[1 0 0 0]  TranslationMethod=None  TranslationCartesianOffset=[0 0 0]  TranslationCartesianOffsetUnits=m  TranslationStandardAxis=+Z  TranslationStandardOffset=0  TranslationStandardOffsetUnits=m  TranslationROffset=0  TranslationROffsetUnits=m  TranslationThetaOffset=0  TranslationThetaOffsetUnits=deg  TranslationZOffset=0  TranslationZOffsetUnits=m
  F : PMIOPort  Side=Right
  B : PMIOPort  Port=2  Side=Left
  connections:
  Transform Steer Axis/RConn1 -- F/RConn1
  B/RConn1 -- Transform HP Wheel/LConn1
  Transform HP Wheel/RConn1 -- Transform Steer Axis/LConn1

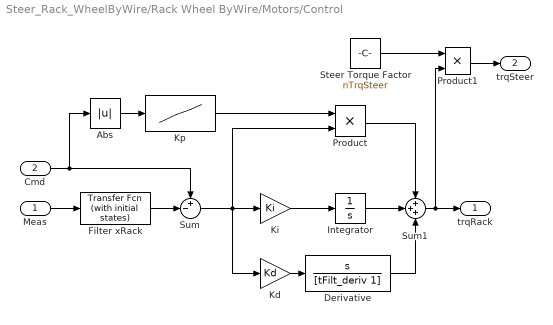
== system Steer_Rack_WheelByWire/Rack Wheel ByWire/Motors/Control ==
  Meas : Inport
  Cmd : Inport  Port=2
  Abs : Abs  ZeroCross=off  SaturateOnIntegerOverflow=off
  Derivative : TransferFcn  Numerator=[1 0]  Denominator=[tFilt_deriv 1]
  Filter xRack : simulink_extras/Additional Linear/Transfer Fcn (with initial states)  N=[1]  D=[tFilt_xRack 1]  X0=0
  Integrator : Integrator
  Kd : Gain  Gain=Kd
  Ki : Gain  Gain=Ki
  Kp : Lookup_n-D  NumberOfTableDimensions=1  BreakpointsForDimension1=Kp_breakpoints  Table=Kp_values  InternalRulePriority=Speed  RndMeth=Simplest
  Product : Product
  Product1 : Product
  Steer Torque Factor : Constant  Value=nTrqSteer
  Sum : Sum  Inputs=+-|
  Sum1 : Sum  Inputs=+++
  trqRack : Outport
  trqSteer : Outport  Port=2
  wires:
  Sum1/1 -> trqRack/1, Product1/2
  Product1/1 -> trqSteer/1
  Steer Torque Factor/1 -> Product1/1
  Abs/1 -> Kp/1
  Kp/1 -> Product/1
  Filter xRack/1 -> Sum/2
  Derivative/1 -> Sum1/3
  Kd/1 -> Derivative/1
  Product/1 -> Sum1/1
  Ki/1 -> Integrator/1
  Integrator/1 -> Sum1/2
  Sum/1 -> Kd/1, Product/2, Ki/1
  Meas/1 -> Filter xRack/1
  Cmd/1 -> Abs/1, Sum/1

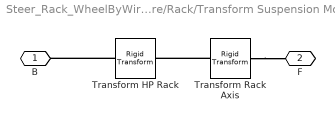
== system Steer_Rack_WheelByWire/Rack Wheel ByWire/Rack/Transform Suspension Mount ==
  Transform HP Rack : sm_lib/Frames and Transforms/Rigid Transform  RotationMethod=None  FollAlignAxisA=+X  BaseAlignAxisA=+Y  FollAlignAxisB=+Y  BaseAlignAxisB=+Z  RotationStandardAxis=+Z  RotationAngle=0.0  RotationAngleUnits=deg  RotationArbitraryAxis=[0 0 1]  RotationSequenceAxes=FollowerAxes  RotationSequence=XYX  RotationSequenceAngles=[0 0 0]  RotationSequenceAnglesUnits=deg  RotationMatrix=[1 0 0; 0 1 0; 0 0 1]  Quaternion=[1 0 0 0]  TranslationMethod=Cartesian  TranslationCartesianOffset=hp_mt_rack  TranslationCartesianOffsetUnits=m  TranslationStandardAxis=+Z  TranslationStandardOffset=0  TranslationStandardOffsetUnits=m  TranslationROffset=0  TranslationROffsetUnits=m  TranslationThetaOffset=0  TranslationThetaOffsetUnits=deg  TranslationZOffset=0  TranslationZOffsetUnits=m
  Transform Rack Axis : sm_lib/Frames and Transforms/Rigid Transform  RotationMethod=AlignedAxes  FollAlignAxisA=+Y  BaseAlignAxisA=-Z  FollAlignAxisB=+X  BaseAlignAxisB=+X  RotationStandardAxis=+Z  RotationAngle=0  RotationAngleUnits=deg  RotationArbitraryAxis=[0 0 1]  RotationSequenceAxes=FollowerAxes  RotationSequence=XYX  RotationSequenceAngles=[0 0 0]  RotationSequenceAnglesUnits=deg  RotationMatrix=[0 0 -1;0 1 0;1 0 0]  Quaternion=[1 0 0 0]  TranslationMethod=None  TranslationCartesianOffset=[0 0 0]  TranslationCartesianOffsetUnits=m  TranslationStandardAxis=+Z  TranslationStandardOffset=0  TranslationStandardOffsetUnits=m  TranslationROffset=0  TranslationROffsetUnits=m  TranslationThetaOffset=0  TranslationThetaOffsetUnits=deg  TranslationZOffset=0  TranslationZOffsetUnits=m
  B : PMIOPort  Side=Left
  F : PMIOPort  Port=2  Side=Right
  connections:
  Transform Rack Axis/RConn1 -- F/RConn1
  Transform HP Rack/LConn1 -- B/RConn1
  Transform Rack Axis/LConn1 -- Transform HP Rack/RConn1
